simulink model "Partie5_QPSK"  (R2026b)
settings: Solver=FixedStepDiscrete  StopTime=Nbits*Tb
undefined symbols (not defined in the file): graine, graine_bruit, p1, Tb, variance_bruit_qpsk
libraries: simulink x2
settings Model: Creator=WORLD COMPUTERS  LastModifiedBy=WORLD COMPUTERS

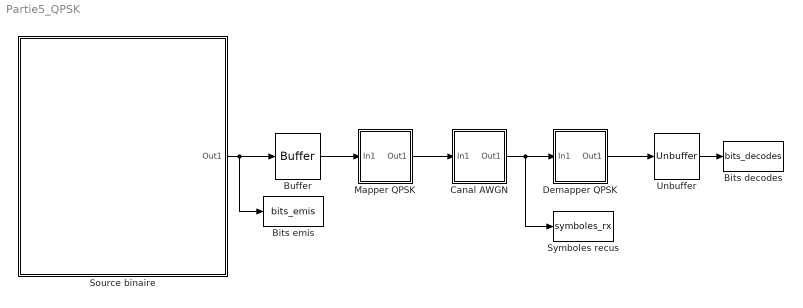
== system Partie5_QPSK ==
  Bits decodes : ToWorkspace  VariableName=bits_decodes  SampleTime=-1
  Bits emis : ToWorkspace  VariableName=bits_emis  SampleTime=-1
  Buffer : Buffer  N=2
  Canal AWGN : Subsystem
  Demapper QPSK : Subsystem
  Mapper QPSK : Subsystem
  Source binaire : Subsystem
  Symboles recus : ToWorkspace  VariableName=symboles_rx  SampleTime=-1
  Unbuffer : Unbuffer
  wires:
  Mapper QPSK/1(Out1) -> Canal AWGN/1(In1)
  Source binaire/1(Out1) -> Buffer/1, Bits emis/1
  Buffer/1 -> Mapper QPSK/1(In1)
  Demapper QPSK/1(Out1) -> Unbuffer/1
  Canal AWGN/1(Out1) -> Demapper QPSK/1(In1), Symboles recus/1
  Unbuffer/1 -> Bits decodes/1

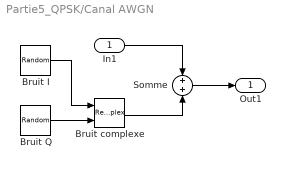
== system Partie5_QPSK/Canal AWGN ==
  In1 : Inport
  Bruit I : RandomNumber  Variance=variance_bruit_qpsk*ones(1,1)  Seed=graine_bruit+(1:1)'  SampleTime=2*Tb
  Bruit Q : RandomNumber  Variance=variance_bruit_qpsk*ones(1,1)  Seed=graine_bruit+100+(1:1)'  SampleTime=2*Tb
  Bruit complexe : RealImagToComplex
  Somme : Sum
  Out1 : Outport
  wires:
  Somme/1 -> Out1/1
  Bruit complexe/1 -> Somme/2
  Bruit Q/1 -> Bruit complexe/2
  Bruit I/1 -> Bruit complexe/1
  In1/1 -> Somme/1

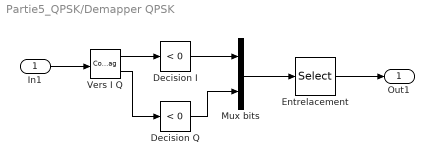
== system Partie5_QPSK/Demapper QPSK ==
  In1 : Inport
  Decision I : simulink/Logic and Bit Operations/Compare To Constant  relop=<  const=0  OutDataTypeStr=boolean
  Decision Q : simulink/Logic and Bit Operations/Compare To Constant  relop=<  const=0  OutDataTypeStr=boolean
  Entrelacement : Selector  InputPortWidth=2  IndexOptions=Index vector (dialog)  Indices="[1  2]"  OutputSizes=1
  Mux bits : Mux  Inputs=2
  Vers I Q : ComplexToRealImag
  Out1 : Outport
  wires:
  Vers I Q/1 -> Decision I/1
  In1/1 -> Vers I Q/1
  Entrelacement/1 -> Out1/1
  Mux bits/1 -> Entrelacement/1
  Decision Q/1 -> Mux bits/2
  Vers I Q/2 -> Decision Q/1
  Decision I/1 -> Mux bits/1

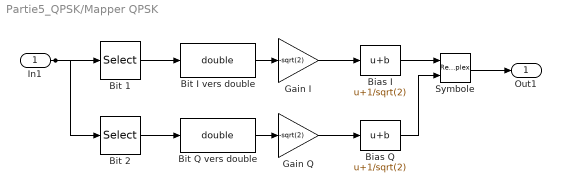
== system Partie5_QPSK/Mapper QPSK ==
  In1 : Inport
  Bias I : Bias  Bias=1/sqrt(2)  SaturateOnIntegerOverflow=off
  Bias Q : Bias  Bias=1/sqrt(2)  SaturateOnIntegerOverflow=off
  Bit 1 : Selector  InputPortWidth=2  IndexOptions=Index vector (dialog)  Indices=[1]  OutputSizes=1
  Bit 2 : Selector  InputPortWidth=2  IndexOptions=Index vector (dialog)  Indices=[2]  OutputSizes=1
  Bit I vers double : DataTypeConversion  OutDataTypeStr=double  SaturateOnIntegerOverflow=off  RndMeth=Floor
  Bit Q vers double : DataTypeConversion  OutDataTypeStr=double  SaturateOnIntegerOverflow=off  RndMeth=Floor
  Gain I : Gain  Gain=-sqrt(2)
  Gain Q : Gain  Gain=-sqrt(2)
  Symbole : RealImagToComplex
  Out1 : Outport
  wires:
  In1/1 -> Bit 1/1, Bit 2/1
  Gain I/1 -> Bias I/1
  Gain Q/1 -> Bias Q/1
  Bit 2/1 -> Bit Q vers double/1
  Bit 1/1 -> Bit I vers double/1
  Bit I vers double/1 -> Gain I/1
  Bias I/1 -> Symbole/1
  Bit Q vers double/1 -> Gain Q/1
  Bias Q/1 -> Symbole/2
  Symbole/1 -> Out1/1

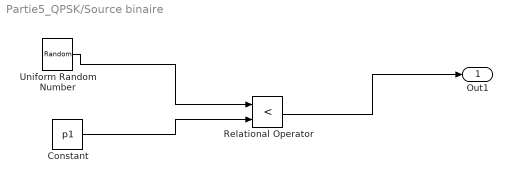
== system Partie5_QPSK/Source binaire ==
  Constant : Constant  Value=p1
  Relational Operator : RelationalOperator  Operator=<  OutDataTypeStr=boolean  RndMeth=Simplest  InputSameDT=off
  Uniform Random Number : UniformRandomNumber  Minimum=0  Seed=graine  SampleTime=Tb
  Out1 : Outport
  wires:
  Relational Operator/1 -> Out1/1
  Constant/1 -> Relational Operator/2
  Uniform Random Number/1 -> Relational Operator/1
